simulink model "test_pol_zero"  (R2024b)
settings: Solver=VariableStepAuto  StartTime=0.0  StopTime=100  RelTol=1e-3
undefined symbols (not defined in the file or in its folder): denP_acc1, denR_acc1, numP_acc1, numR_acc1
settings Model: Creator=razva  LastModifiedBy=razva

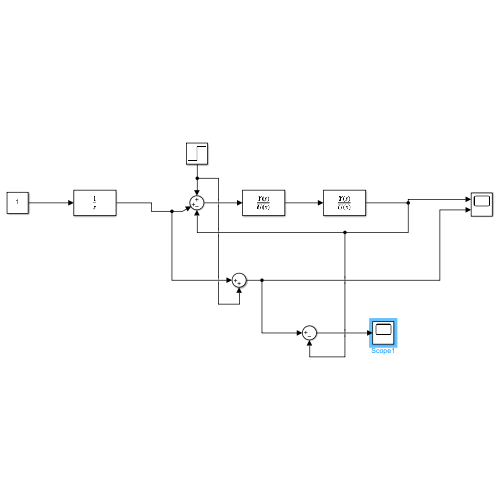
[thumbnail: Simulink's stored preview of the top-level diagram]
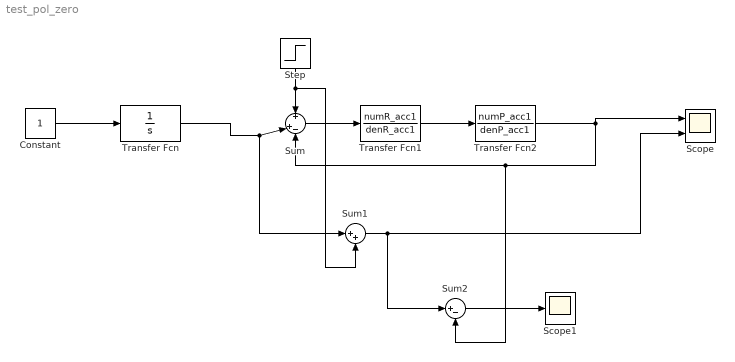
== system test_pol_zero ==
  Constant : Constant
  Scope : Scope  NumInputPorts=2
  Scope1 : Scope
  Step : Step  Time=0  SampleTime=0
  Sum : Sum  Inputs=+|+-
  Sum1 : Sum  Inputs=|++
  Sum2 : Sum  Inputs=|+-
  Transfer Fcn : TransferFcn  Denominator=[1 0]
  Transfer Fcn1 : TransferFcn  Numerator=numR_acc1  Denominator=denR_acc1
  Transfer Fcn2 : TransferFcn  Numerator=numP_acc1  Denominator=denP_acc1
  wires:
  Constant/1 -> Transfer Fcn/1
  Step/1 -> Sum1/2, Sum/1
  Sum/1 -> Transfer Fcn1/1
  Transfer Fcn1/1 -> Transfer Fcn2/1
  Transfer Fcn2/1 -> Sum2/2, Sum/3, Scope/1
  Transfer Fcn/1 -> Sum1/1, Sum/2
  Sum1/1 -> Sum2/1, Scope/2
  Sum2/1 -> Scope1/1
